simulink subsystem "state_estimator"  (R2026a)
settings: Solver=VariableStepAuto
undefined symbols (not defined in the file): DiscIntNeverNeededParam, dRb0_est, P, S, T
PreSaveFcn:
  | defaultToFileBlockNames(bdroot);
settings Model: Creator=kjhaydon  LastModifiedBy=kjhaydon

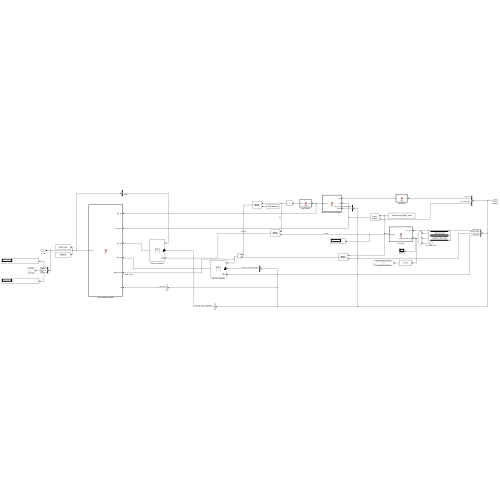
[thumbnail: Simulink's stored preview of the top-level diagram]
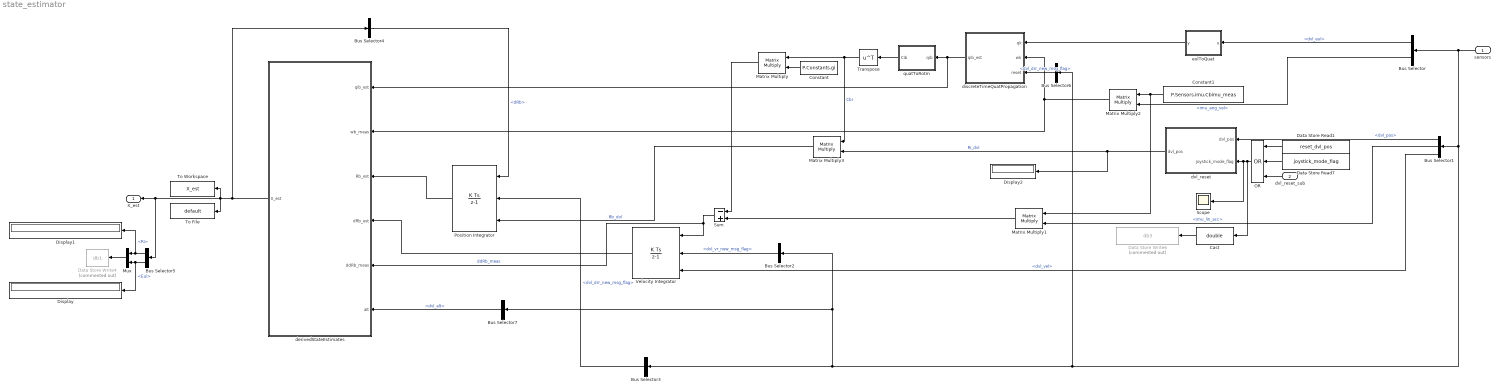
== system state_estimator ==
  sensors : Inport  OutDataTypeStr=Bus: sensor_bus  SampleTime=S.dt_control
  dvl_reset_sub : Inport  Port=2
  Bus Selector : BusSelector  OutputSignals=dvl_eul,imu_ang_vel
  Bus Selector1 : BusSelector  OutputSignals=dvl_pos,imu_lin_acc,dvl_vel
  Bus Selector2 : BusSelector  OutputSignals=dvl_vr_new_msg_flag
  Bus Selector3 : BusSelector  OutputSignals=dvl_drr_new_msg_flag
  Bus Selector4 : BusSelector  OutputSignals=dRb
  Bus Selector5 : BusSelector  OutputSignals=Ri,Eul
  Bus Selector6 : BusSelector  OutputSignals=dvl_drr_new_msg_flag
  Bus Selector7 : BusSelector  OutputSignals=dvl_alt
  Cast : DataTypeConversion  OutDataTypeStr=double  SaturateOnIntegerOverflow=off  RndMeth=Floor
  Constant : Constant  Value=P.Constants.gi
  Constant1 : Constant  Value=P.Sensors.imu.Cbimu_meas
  Data Store Read1 : DataStoreRead  DataStoreName=reset_dvl_pos  IndexOptions=Index vector (dialog)  Indices=1  OutputSizes=1
  Data Store Read7 : DataStoreRead  DataStoreName=joystick_mode_flag  IndexOptions=Index vector (dialog)  Indices=1  OutputSizes=1
  Data Store Write4 : DataStoreWrite  Commented=on  DataStoreName=db1  IndexOptions=Index vector (dialog)  Indices=1  OutputSizes=1
  Data Store Write6 : DataStoreWrite  Commented=on  DataStoreName=db3  IndexOptions=Index vector (dialog)  Indices=1  OutputSizes=1
  Display : Display
  Display1 : Display
  Display2 : Display
  Matrix Multiply{,1..3} (4 alike) : Product  Multiplication=Matrix(*)
  Mux : Mux  Inputs=2
  OR : Logic  Operator=OR  Inputs=3  IconShape=distinctive  AllPortsSameDT=off  OutDataTypeStr=boolean
  Position Integrator : DiscreteIntegrator  ExternalReset=rising  InitialConditionSource=external  InitialCondition=dRb0_est  SampleTime=S.dt_control  ICPrevOutput=DiscIntNeverNeededParam  ICPrevScaledInput=DiscIntNeverNeededParam
  Scope : Scope
      settings: ActiveDisplayYMinimum=-1  ActiveDisplayYMaximum=1  DataLoggingVariableName=ScopeData5
  Sum : Sum  Inputs=-+
  To File : ToFile  Filename=default  MatrixName=X_est  SaveFormat=Timeseries  SampleTime=S.dt_data
  To Workspace : ToWorkspace  VariableName=X_est  SaveFormat=Timeseries  SampleTime=S.dt_data
  Transpose : Math  Operator=transpose
  Velocity Integrator : DiscreteIntegrator  ExternalReset=rising  InitialConditionSource=external  InitialCondition=dRb0_est  SampleTime=S.dt_control  ICPrevOutput=DiscIntNeverNeededParam  ICPrevScaledInput=DiscIntNeverNeededParam
  derivedStateEstimates : MATLAB Function  TreatAsAtomicUnit=on
  discreteTimeQuatPropagation : MATLAB Function  TreatAsAtomicUnit=on
  dvl_reset : MATLAB Function  TreatAsAtomicUnit=on
  eulToQuat : MATLAB Function  TreatAsAtomicUnit=on
  quatToRotm : MATLAB Function  TreatAsAtomicUnit=on
  X_est : Outport  SampleTime=S.dt_control
  wires:
  sensors/1 -> Bus Selector1/1, Bus Selector7/1, Bus Selector2/1, Bus Selector3/1, Bus Selector6/1, Bus Selector/1
  eulToQuat/1(y) -> discreteTimeQuatPropagation/1(qk)
  Velocity Integrator/1 -> derivedStateEstimates/4(dRb_est)
  discreteTimeQuatPropagation/1(qib_est) -> quatToRotm/1(qib), derivedStateEstimates/1(qib_est)
  Position Integrator/1 -> derivedStateEstimates/3(Rb_est)
  quatToRotm/1(Cib) -> Transpose/1
  Constant/1 -> Matrix Multiply/2
  Transpose/1 -> Matrix Multiply3/1, Matrix Multiply/1  "Cbi"
  Matrix Multiply/1 -> Sum/1
  Sum/1 -> Velocity Integrator/1, derivedStateEstimates/5(ddRb_meas)  "ddRb_meas"
  Bus Selector1/2 -> Matrix Multiply1/2  "<imu_lin_acc>"
  Matrix Multiply1/1 -> Sum/2
  Bus Selector/2 -> Matrix Multiply2/2  "<imu_ang_vel>"
  Bus Selector1/1 -> dvl_reset/1("dvl_pos ")  "<dvl_pos>"
  Bus Selector/1 -> eulToQuat/1(u)  "<dvl_eul>"
  Bus Selector6/1 -> discreteTimeQuatPropagation/3(reset)  "<dvl_drr_new_msg_flag>"
  Bus Selector2/1 -> Velocity Integrator/2  "<dvl_vr_new_msg_flag>"
  Bus Selector3/1 -> Position Integrator/2  "<dvl_drr_new_msg_flag>"
  Bus Selector1/3 -> Velocity Integrator/3  "<dvl_vel>"
  derivedStateEstimates/1(X_est) -> Bus Selector5/1, X_est/1, To File/1, To Workspace/1, Bus Selector4/1
  Bus Selector4/1 -> Position Integrator/1  "<dRb>"
  Bus Selector5/1 -> Mux/1, Display1/1  "<Ri>"
  Bus Selector5/2 -> Mux/2, Display/1  "<Eul>"
  Mux/1 -> Data Store Write4/1
  Cast/1 -> Data Store Write6/1
  OR/1 -> dvl_reset/2(joystick_mode_flag), Scope/1, Cast/1
  Data Store Read1/1 -> OR/1
  dvl_reset_sub/1 -> OR/3
  Constant1/1 -> Matrix Multiply2/1, Matrix Multiply1/1
  Matrix Multiply2/1 -> derivedStateEstimates/2(wb_meas), discreteTimeQuatPropagation/2(wk)
  dvl_reset/1(dvl_pos) -> Display2/1, Matrix Multiply3/2  "Ri_dvl"
  Matrix Multiply3/1 -> Position Integrator/3  "Rb_dvl"
  Data Store Read7/1 -> OR/2
  Bus Selector7/1 -> derivedStateEstimates/6(alt)  "<dvl_alt>"

== matlab function state_estimator/derivedStateEstimates ==
  settings: updateMethod=DISCRETE  sampleTime=S.dt_control
  data: qib_est input; X_est output Bus: X_bus; wb_meas input; Rb_est input; dRb_est input; ddRb_meas input; alt input
function X_est = fcn(qib_est, wb_meas, Rb_est, dRb_est, ddRb_meas, alt)

X_est = derivedStateEstimates(qib_est, wb_meas, Rb_est, dRb_est, ddRb_meas, alt);

== matlab function state_estimator/discreteTimeQuatPropagation ==
  settings: updateMethod=DISCRETE  sampleTime=S.dt_control
  data: qk input; qib_est output; wk input; reset input; T parameter; S parameter
function qib_est = fcn(qk, wk, reset, T, S)

dt_control = S.dt_control;
q0_est = T.q0_est;

qib_est = discreteTimeQuatPropagation(qk, wk, reset, q0_est, dt_control);

== matlab function state_estimator/dvl_reset ==
  data: dvl_pos input; joystick_mode_flag input; dvl_pos output
function dvl_pos = fcn(dvl_pos, joystick_mode_flag)
%{
Reset the dvl position used for the state estimator.
%}
persistent offset;
persistent prior_flag;

if (isempty(offset))
    offset = [0;0;0];
end
if (isempty(prior_flag))
    prior_flag = true;
end

%switch on falling edge
if((prior_flag && ~joystick_mode_flag))
    offset = dvl_pos;
end

dvl_pos = dvl_pos - offset;
prior_flag = joystick_mode_flag;

== matlab function state_estimator/eulToQuat ==
  data: u input; y output
function y = fcn(u)

y = eulToQuat(u);

== matlab function state_estimator/quatToRotm ==
  data: qib input; Cib output
function Cib = fcn(qib)

Cib = quatToRotm(qib);
